simulink model "RobustFormationControl_FractionalModel_under_Dis"  (R2023a)
settings: Solver=ode3  StartTime=0.0  StopTime=30  FixedStep=0.0001  RelTol=1e-3
InitFcn:
  | % close all;
  | % clear all;
  | % clc;
  | % System & Qaudrotor Parameters
  | %==============================
  | m = 0.486;                                         % Quadrotor Mass ( kg )
  | 
  | L = 0.25;                                         % Length of the arm ( m )
  | % L = 0.25;                                         % Length of the arm ( m )
  | 
  | Ixx = 4.856e-03; Iyy = 4.856e-03; Izz = 8.801e-03; % The moments of inertia around x,y and z axes respectively ( kg.m^2 )
  | % Ixx = 3.8278e-03; Iyy = 3.8278e-03; Izz = 7.6566e-03; % The moments of inertia around x,y and z axes respectively ( kg.m^2 )
  | 
  | Jr = 2.8385e-5;                                            % The inertia moment of rotor ( kg.m^2 )
  | % Jr = 0;
  | 
  | % Kx=5.5670e-4;
  | % Ky=5.5670e-4;
  | % Kz=6.3540e-4;
  | % kx=0.032;
  | % ky=0.032;
  | % kz=0.048;
  | Kfx = 5.5670e-4; Kfy = 5.5670e-4; Kfz = 6.3540e-4;% The Rotational drag cofficients ( N/rad/s )
  | 
  | % Ktx = 0.032; Kty = 0.032; Ktz = 0.048;               % The linear drag coefficients in x, y, z respectively ( N/m/s )
  | Ktx = 5.5670e-4; Kty =5.5670e-4; Ktz = 6.3540e-4;               % The linear drag coefficients in x, y, z respectively ( N/m/s )
  | 
  | b = 2.923e-05;                                      % The lift coefficient
  | % b = 2.9842e-05;                                      % The lift coefficient
  | 
  | d = 1.12e-06;                                       % The drag coefficient
  | % d = 3.2320e-07;                                       % The drag coefficient
  | 
  | g = 9.81;                                          % The acceleration due to gravity ( m/s^2 )
  | 
  | %-------- The Coefficients of Non-linear Equations of Quadrotor ( Page 11) -------
  | %--------------------------------------------------------------------------------
  | % Rotational Equations
  | %=====================
  | % Coefficients in ( eq1 ) >>..
  | a1 = (Iyy - Izz)/Ixx;
  | b1 = - Jr/Ixx;
  | c1 = - Kfx/Ixx;
  | d1 = L/Ixx;
  | 
  | % Coefficients in ( eq2 ) >>..
  | a2 = (Izz - Ixx)/Iyy;
  | b2 = Jr/Iyy;
  | c2 = - Kfy/Iyy;
  | d2 = L/Iyy;
  | 
  | % Coefficients in ( eq3 ) >>..
  | a3 = (Ixx - Iyy)/Izz;
  | b3 = - Kfz/Izz;
  | c3 = 1/Izz;
  | % c3 = d/Izz;
  | 
  | % Translational Equations
  | %========================
  | % Coefficients in ( eq4 ) >>..
  | ... (+151 lines)
libraries: fod x135, eeStairGenerator x5
(part 5 of 10)

== system RobustFormationControl_FractionalModel_under_Dis/Fractional Leader with four followers/Follower 4 System/Follower 2 Quadrotor Model/Control Module1/Subsystem1 ==
  x1 : Inport
  x2 : Inport  Port=2
  x3 : Inport  Port=3
  x4 : Inport  Port=4
  x5 : Inport  Port=5
  x6 : Inport  Port=6
  x7 : Inport  Port=7
  x8 : Inport  Port=8
  x9 : Inport  Port=9
  x10 : Inport  Port=10
  x11 : Inport  Port=11
  x12 : Inport  Port=12
  xd1 : Inport  Port=13
  xd2 : Inport  Port=14
  xd3 : Inport  Port=15
  xd4 : Inport  Port=16
  xd5 : Inport  Port=17
  xd6 : Inport  Port=18
  xL : Inport  Port=19
  dX : Inport  Port=20
  yL : Inport  Port=21
  dY : Inport  Port=22
  zL : Inport  Port=23
  dZ : Inport  Port=24
  Subsystem : Subsystem
  Subsystem1 : Subsystem
  Subsystem2 : Subsystem
  Subsystem3 : Subsystem
  Subsystem4 : Subsystem
  Subsystem6 : Subsystem
  S2 : Outport  VectorParamsAs1DForOutWhenUnconnected=off
  S4 : Outport  Port=2  VectorParamsAs1DForOutWhenUnconnected=off
  S6 : Outport  Port=3  VectorParamsAs1DForOutWhenUnconnected=off
  S8 : Outport  Port=4  VectorParamsAs1DForOutWhenUnconnected=off
  S10 : Outport  Port=5  VectorParamsAs1DForOutWhenUnconnected=off
  S12 : Outport  Port=6  VectorParamsAs1DForOutWhenUnconnected=off
  wires:
  x1/1 -> [x1]
  x2/1 -> [x2]
  x3/1 -> [x3]
  x4/1 -> [x4]
  x5/1 -> [x5]
  x6/1 -> [x6]
  x7/1 -> [x7]
  x8/1 -> [x8]
  x9/1 -> [x9]
  x10/1 -> [x10]
  x11/1 -> [x11]
  x12/1 -> [x12]
  xd1/1 -> [xd1]
  dY/1 -> [dY]
  xd2/1 -> [xd2]
  xd3/1 -> [xd3]
  xd4/1 -> [xd4]
  xd5/1 -> [xd5]
  xd6/1 -> [xd6]
  xL/1 -> [xL]
  dX/1 -> [dX]
  yL/1 -> [yL]
  zL/1 -> [zL]
  dZ/1 -> [dZ]
  [x1] -> Subsystem/1(x1)
  [xd1] -> Subsystem/2(xd1)
  [x2] -> Subsystem/3(x2)
  [xd2] -> Subsystem/4(xd2)
  Subsystem/1(S2) -> S2/1
  [xd4] -> Subsystem6/4(xd4)
  [x3] -> Subsystem6/1(x3)
  [x4] -> Subsystem6/3(x4)
  [xd3] -> Subsystem6/2(xd3)
  [xd6] -> Subsystem1/4(xd6)
  [x5] -> Subsystem1/1(x5)
  [x6] -> Subsystem1/3(x6)
  [xd5] -> Subsystem1/2(xd5)
  Subsystem6/1(S4) -> S4/1
  Subsystem1/1(S6) -> S6/1
  [x9] -> Subsystem2/2(x9)
  [x10] -> Subsystem2/3(x10)
  [yL] -> Subsystem2/1(yL)
  [dY] -> Subsystem2/4(dY)
  Subsystem2/1(S10) -> S10/1
  [zL] -> Subsystem4/1(zL)
  [x8] -> Subsystem3/3(x8)
  Subsystem4/1(S12) -> S12/1
  [x12] -> Subsystem4/3(x12)
  Subsystem3/1(S8) -> S8/1
  [dZ] -> Subsystem4/4(dZ)
  [x11] -> Subsystem4/2(x11)
  [x7] -> Subsystem3/2(x7)
  [dX] -> Subsystem3/4(dX)
  [xL] -> Subsystem3/1(xL)

== system RobustFormationControl_FractionalModel_under_Dis/Fractional Leader with four followers/Follower 4 System/Follower 2 Quadrotor Model/Control Module1/Subsystem10 ==
  x1 : Inport
  x3 : Inport  Port=2
  x11 : Inport  Port=3
  x12 : Inport  Port=4
  zL : Inport  Port=5
  dZ : Inport  Port=6
  S12 : Inport  Port=7
  Constant1 : Constant
  Divide1 : Product  Inputs=*/
  Divide2 : Product  Inputs=**  RndMeth=Zero  SaturateOnIntegerOverflow=on
  Gain : Gain  Commented=on  Gain=b6
  Product1 : Product
  Product2 : Product
  Subsystem : Subsystem
  Subsystem1 : Subsystem
  Subsystem2 : Subsystem
  Sum2 : Sum  Inputs=+++
  Trigonometric Function1 : Trigonometry  Operator=cos
  Trigonometric Function2 : Trigonometry  Operator=cos
  U1 : Outport  VectorParamsAs1DForOutWhenUnconnected=off
  wires:
  S12/1 -> [S12]
  dZ/1 -> [dZ]
  zL/1 -> [zL]
  x3/1 -> [x3]
  Sum2/1 -> Product2/2
  Product2/1 -> U1/1
  x11/1 -> [x11]
  x12/1 -> [x12]
  x1/1 -> [x1]
  [x11] -> Subsystem/2(x11)
  [x12] -> Subsystem1/1(x12)
  [zL] -> Subsystem1/2(zL)
  [zL] -> Subsystem/1(zL)
  [dZ] -> Subsystem/4(dZ)
  [x12] -> Subsystem/3(x12)
  [S12] -> Subsystem/5(S12)
  [x11] -> Subsystem2/2(x11)
  [S12] -> Subsystem2/5(S12)
  [x12] -> Subsystem2/3(x12)
  [zL] -> Subsystem2/1(zL)
  [dZ] -> Subsystem2/4(dZ)
  Subsystem/1(D2) -> Sum2/2
  Subsystem2/1(D3) -> Sum2/3
  Subsystem1/1(D1) -> Sum2/1
  Divide1/1 -> Product2/1
  Constant1/1 -> Divide1/1
  Trigonometric Function2/1 -> Product1/2
  Trigonometric Function1/1 -> Product1/1
  Divide2/1 -> Divide1/2
  Product1/1 -> Divide2/2
  [x1] -> Trigonometric Function1/1
  [x3] -> Trigonometric Function2/1
  [b6D] -> Divide2/1
  [dZ] -> Subsystem1/3(dZ)

== system RobustFormationControl_FractionalModel_under_Dis/Fractional Leader with four followers/Follower 4 System/Follower 2 Quadrotor Model/Control Module1/Subsystem2 ==
  U1 : Inport
  x9 : Inport  Port=2
  x10 : Inport  Port=3
  yL : Inport  Port=4
  dY : Inport  Port=5
  S10 : Inport  Port=6
  Constant1 : Constant
  Divide1 : Product  Inputs=*/
  Divide2 : Product  Inputs=**  RndMeth=Zero  SaturateOnIntegerOverflow=on
  Gain1 : Gain  Commented=on  Gain=b4
  Product2 : Product
  Subsystem3 : Subsystem
  Subsystem4 : Subsystem
  Subsystem5 : Subsystem
  Sum1 : Sum  Inputs=+++
  Uy : Outport  VectorParamsAs1DForOutWhenUnconnected=off
  wires:
  S10/1 -> [S10]
  dY/1 -> [dY]
  yL/1 -> [yL]
  Product2/1 -> Uy/1
  x9/1 -> [x9]
  x10/1 -> [x10]
  U1/1 -> [U1]
  Divide1/1 -> Product2/1
  Constant1/1 -> Divide1/1
  [b5D] -> Divide2/1
  [U1] -> Divide2/2
  Divide2/1 -> Divide1/2
  [dY] -> Subsystem4/3(dY)
  [dY] -> Subsystem3/4(dY)
  Subsystem4/1(D1) -> Sum1/1
  Subsystem5/1(D3) -> Sum1/3
  [yL] -> Subsystem5/1(yL)
  Subsystem3/1(D2) -> Sum1/2
  [dY] -> Subsystem5/4(dY)
  [x9] -> Subsystem3/2(x9)
  [yL] -> Subsystem3/1(yL)
  [yL] -> Subsystem4/2(yL)
  [S10] -> Subsystem3/5(S10)
  [x9] -> Subsystem5/2(x9)
  [x10] -> Subsystem5/3(x10)
  [x10] -> Subsystem4/1(x10)
  [x10] -> Subsystem3/3(x10)
  [S10] -> Subsystem5/5(S10)
  Sum1/1 -> Product2/2

== system RobustFormationControl_FractionalModel_under_Dis/Fractional Leader with four followers/Follower 4 System/Follower 2 Quadrotor Model/Control Module1/Subsystem4 ==
  x1 : Inport
  x2 : Inport  Port=2
  x4 : Inport  Port=3
  x6 : Inport  Port=4
  xd1 : Inport  Port=5
  xd2 : Inport  Port=6
  S2 : Inport  Port=7
  Omega : Inport  Port=8
  Constant : Constant
  Constant3 : Constant  Value=d1
  Derivative : Derivative
  Divide : Product  Inputs=*/
  Product2 : Product
  Subsystem : Subsystem
  Subsystem1 : Subsystem
  Subsystem2 : Subsystem
  Sum2 : Sum  Inputs=+++
  U2 : Outport  VectorParamsAs1DForOutWhenUnconnected=off
  wires:
  Constant/1 -> Divide/1
  Constant3/1 -> Divide/2
  S2/1 -> [S2]
  xd2/1 -> [xd2], Derivative/1
  Derivative/1 -> [xdDot2]
  xd1/1 -> [xd1]
  x2/1 -> [x2]
  Sum2/1 -> Product2/2
  Divide/1 -> Product2/1
  Product2/1 -> U2/1
  x4/1 -> [x4]
  x6/1 -> [x6]
  x1/1 -> [x1]
  [x1] -> Subsystem/1(x1)
  [x4] -> Subsystem1/1(x4)
  [x6] -> Subsystem1/2(x6)
  [x2] -> Subsystem1/3(x2)
  Omega/1 -> Subsystem1/4(Omega)
  [xdDot2] -> Subsystem1/5(xd2)
  [xd1] -> Subsystem/2(xd1)
  [xd2] -> Subsystem/4(xd2)
  [x2] -> Subsystem/3(x2)
  [S2] -> Subsystem/5(S2)
  [xd1] -> Subsystem2/2(xd1)
  [S2] -> Subsystem2/5(S2)
  [x2] -> Subsystem2/3(x2)
  [x1] -> Subsystem2/1(x1)
  [xd2] -> Subsystem2/4(xd2)
  Subsystem1/1(D1) -> Sum2/1
  Subsystem/1(D2) -> Sum2/2
  Subsystem2/1(D3) -> Sum2/3

== system RobustFormationControl_FractionalModel_under_Dis/Fractional Leader with four followers/Follower 4 System/Follower 2 Quadrotor Model/Control Module1/Subsystem5 ==
  x5 : Inport
  x2 : Inport  Port=2
  x4 : Inport  Port=3
  x6 : Inport  Port=4
  xd5 : Inport  Port=5
  xd6 : Inport  Port=6
  S6 : Inport  Port=7
  Constant : Constant
  Constant3 : Constant  Value=c3
  Derivative : Derivative
  Divide : Product  Inputs=*/
  Product2 : Product
  Subsystem : Subsystem
  Subsystem1 : Subsystem
  Subsystem2 : Subsystem
  Sum2 : Sum  Inputs=+++
  U4 : Outport  VectorParamsAs1DForOutWhenUnconnected=off
  wires:
  Constant/1 -> Divide/1
  Constant3/1 -> Divide/2
  S6/1 -> [S6]
  xd6/1 -> [xd6], Derivative/1
  Derivative/1 -> [xdDot6]
  xd5/1 -> [xd5]
  x2/1 -> [x2]
  Sum2/1 -> Product2/2
  Divide/1 -> Product2/1
  Product2/1 -> U4/1
  x4/1 -> [x4]
  x6/1 -> [x6]
  x5/1 -> [x5]
  [x5] -> Subsystem/1(x5)
  [x4] -> Subsystem1/1(x4)
  [x6] -> Subsystem1/2(x6)
  [x2] -> Subsystem1/3(x2)
  [xdDot6] -> Subsystem1/4(xd6)
  [xd5] -> Subsystem/2(xd5)
  [xd6] -> Subsystem/4(xd6)
  [x6] -> Subsystem/3(x6)
  [S6] -> Subsystem/5(S4)
  [xd5] -> Subsystem2/2(xd5)
  [S6] -> Subsystem2/5(S6)
  [x6] -> Subsystem2/3(x6)
  [x5] -> Subsystem2/1(x5)
  [xd6] -> Subsystem2/4(xd6)
  Subsystem/1(D2) -> Sum2/2
  Subsystem2/1(D3) -> Sum2/3
  Subsystem1/1(D1) -> Sum2/1

== system RobustFormationControl_FractionalModel_under_Dis/Fractional Leader with four followers/Follower 4 System/Follower 2 Quadrotor Model/Control Module1/Subsystem6 ==
  U1 : Inport
  x7 : Inport  Port=2
  x8 : Inport  Port=3
  xL : Inport  Port=4
  dX : Inport  Port=5
  S8 : Inport  Port=6
  Constant1 : Constant
  Divide1 : Product  Inputs=*/
  Divide2 : Product  Inputs=**  RndMeth=Zero  SaturateOnIntegerOverflow=on
  Gain1 : Gain  Commented=on  Gain=b4
  Product2 : Product
  Subsystem3 : Subsystem
  Subsystem4 : Subsystem
  Subsystem5 : Subsystem
  Sum1 : Sum  Inputs=+++
  Ux : Outport  VectorParamsAs1DForOutWhenUnconnected=off
  wires:
  S8/1 -> [S8]
  dX/1 -> [dX]
  xL/1 -> [xL]
  Product2/1 -> Ux/1
  x7/1 -> [x7]
  x8/1 -> [x8]
  U1/1 -> [U1]
  Divide1/1 -> Product2/1
  Constant1/1 -> Divide1/1
  [b4D] -> Divide2/1
  [U1] -> Divide2/2
  Divide2/1 -> Divide1/2
  [dX] -> Subsystem4/3(dX)
  [dX] -> Subsystem3/4(dX)
  Subsystem4/1(D1) -> Sum1/1
  Subsystem5/1(D3) -> Sum1/3
  [xL] -> Subsystem5/1(xL)
  Subsystem3/1(D2) -> Sum1/2
  [dX] -> Subsystem5/4(dX)
  [x7] -> Subsystem3/2(x7)
  [xL] -> Subsystem3/1(xL)
  [xL] -> Subsystem4/2(xL)
  [S8] -> Subsystem3/5(S8)
  [x7] -> Subsystem5/2(x7)
  [x8] -> Subsystem5/3(x8)
  [x8] -> Subsystem4/1(x8)
  [x8] -> Subsystem3/3(x8)
  [S8] -> Subsystem5/5(S8)
  Sum1/1 -> Product2/2

== system RobustFormationControl_FractionalModel_under_Dis/Fractional Leader with four followers/Follower 4 System/Follower 2 Quadrotor Model/Control Module1/Subsystem8 ==
  x3 : Inport
  x2 : Inport  Port=2
  x4 : Inport  Port=3
  x6 : Inport  Port=4
  xd3 : Inport  Port=5
  xd4 : Inport  Port=6
  S4 : Inport  Port=7
  Omega : Inport  Port=8
  Constant : Constant
  Constant3 : Constant  Value=d2
  Derivative : Derivative
  Divide : Product  Inputs=*/
  Product2 : Product
  Subsystem : Subsystem
  Subsystem1 : Subsystem
  Subsystem2 : Subsystem
  Sum2 : Sum  Inputs=+++
  U3 : Outport  VectorParamsAs1DForOutWhenUnconnected=off
  wires:
  Constant/1 -> Divide/1
  Constant3/1 -> Divide/2
  S4/1 -> [S4]
  xd4/1 -> [xd4], Derivative/1
  Derivative/1 -> [xdDot4]
  xd3/1 -> [xd3]
  x2/1 -> [x2]
  Sum2/1 -> Product2/2
  Divide/1 -> Product2/1
  Product2/1 -> U3/1
  x4/1 -> [x4]
  x6/1 -> [x6]
  x3/1 -> [x3]
  [x3] -> Subsystem/1(x3)
  [x4] -> Subsystem1/1(x4)
  [x6] -> Subsystem1/2(x6)
  [x2] -> Subsystem1/3(x2)
  Omega/1 -> Subsystem1/4(Omega)
  [xdDot4] -> Subsystem1/5(xd4)
  [xd3] -> Subsystem/2(xd3)
  [xd4] -> Subsystem/4(xd4)
  [x4] -> Subsystem/3(x4)
  [S4] -> Subsystem/5(S4)
  [xd3] -> Subsystem2/2(xd3)
  [S4] -> Subsystem2/5(S4)
  [x4] -> Subsystem2/3(x4)
  [x3] -> Subsystem2/1(x3)
  [xd4] -> Subsystem2/4(xd4)
  Subsystem/1(D2) -> Sum2/2
  Subsystem2/1(D3) -> Sum2/3
  Subsystem1/1(D1) -> Sum2/1

== system RobustFormationControl_FractionalModel_under_Dis/Fractional Leader with four followers/Follower 4 System/Follower 2 Quadrotor Model/Quadrotor Dynamic System/Rotational System ==
  U2 : Inport
  U3 : Inport  Port=2
  U4 : Inport  Port=3
  Omega : Inport  Port=4
  Equation1 : Subsystem
  Equation2 : Subsystem
  Equation3 : Subsystem
  Phi or x1 : Outport  VectorParamsAs1DForOutWhenUnconnected=off
  Theta or x3 : Outport  Port=2  VectorParamsAs1DForOutWhenUnconnected=off
  Psi or x5 : Outport  Port=3  VectorParamsAs1DForOutWhenUnconnected=off
  x2 : Outport  Port=4  VectorParamsAs1DForOutWhenUnconnected=off
  x4 : Outport  Port=5  VectorParamsAs1DForOutWhenUnconnected=off
  x6 : Outport  Port=6  VectorParamsAs1DForOutWhenUnconnected=off
  wires:
  Equation1/1(x1 = Phi) -> Phi or x1/1
  Equation3/1(x5 =Psi) -> Psi or x5/1
  U2/1 -> Equation1/3(U2)
  U3/1 -> Equation2/3(U3)
  Equation3/2(x6) -> Equation2/2(x6), x6/1, Equation1/2(x6)
  Equation2/1(x3 =Theta) -> Theta or x3/1
  U4/1 -> Equation3/3(U4)
  Omega/1 -> Equation2/4(Omega), Equation1/4(Omega)
  Equation1/2(x2) -> x2/1, Equation2/1(x2), Equation3/1(x2)
  Equation2/2(x4) -> x4/1, Equation3/2(x4), Equation1/1(x4)

== system RobustFormationControl_FractionalModel_under_Dis/Fractional Leader with four followers/Follower 4 System/Follower 2 Quadrotor Model/Quadrotor Dynamic System/Translational System ==
  U1 : Inport
  Ux : Inport  Port=2
  Uy : Inport  Port=3
  x1 : Inport  Port=4
  x3 : Inport  Port=5
  Equation4 : Subsystem
  Equation5 : Subsystem
  Equation6 : Subsystem
  x or x7 : Outport  VectorParamsAs1DForOutWhenUnconnected=off
  y or x9 : Outport  Port=2  VectorParamsAs1DForOutWhenUnconnected=off
  z or x11 : Outport  Port=3  VectorParamsAs1DForOutWhenUnconnected=off
  xdot or x8 : Outport  Port=4  VectorParamsAs1DForOutWhenUnconnected=off
  ydot or x10 : Outport  Port=5  VectorParamsAs1DForOutWhenUnconnected=off
  zdot or x12 : Outport  Port=6  VectorParamsAs1DForOutWhenUnconnected=off
  wires:
  Ux/1 -> Equation4/2(Ux)
  Uy/1 -> Equation5/2(Uy)
  x1/1 -> Equation6/2(x1)
  x3/1 -> Equation6/3(x3)
  Equation5/1(x9 = y) -> y or x9/1
  Equation6/1(x11 = z) -> z or x11/1
  Equation4/1(x7 = x) -> x or x7/1
  U1/1 -> Equation6/1(U1), Equation5/1(U1), Equation4/1(U1)
  Equation4/2(x8 = xdot) -> xdot or x8/1
  Equation5/2(x10 = ydot) -> ydot or x10/1
  Equation6/2(x12 = zdot) -> zdot or x12/1

== system RobustFormationControl_FractionalModel_under_Dis/Fractional Leader with four followers/Fractional Model of the Leader/Fractional Model/Control Module1/Desired System ==
  ft : Inport
  Derivative : Derivative
  Derivative1 : Derivative
  Derivative2 : Derivative
  Desired Values : Subsystem
  Fractional operator{,1..8} (9 alike) : fod/Fractional operator  Tag=Fractional operator  K=1  gam=0.5  ww=[0.001, 1000]  n=5
      settings: SourceProductName=FOMCON Toolbox
  xd1 : Outport  VectorParamsAs1DForOutWhenUnconnected=off
  xd2 : Outport  Port=2  VectorParamsAs1DForOutWhenUnconnected=off
  xd3 : Outport  Port=3  VectorParamsAs1DForOutWhenUnconnected=off
  xd4 : Outport  Port=4  VectorParamsAs1DForOutWhenUnconnected=off
  xd5 : Outport  Port=5  VectorParamsAs1DForOutWhenUnconnected=off
  xd6 : Outport  Port=6  VectorParamsAs1DForOutWhenUnconnected=off
  xfd7 : Outport  Port=7  VectorParamsAs1DForOutWhenUnconnected=off
  xfd8 : Outport  Port=8  VectorParamsAs1DForOutWhenUnconnected=off
  xfd9 : Outport  Port=9  VectorParamsAs1DForOutWhenUnconnected=off
  xfd10 : Outport  Port=10  VectorParamsAs1DForOutWhenUnconnected=off
  xfd11 : Outport  Port=11  VectorParamsAs1DForOutWhenUnconnected=off
  xfd12 : Outport  Port=12  VectorParamsAs1DForOutWhenUnconnected=off
  xfd13 : Outport  Port=13  VectorParamsAs1DForOutWhenUnconnected=off
  xfd14 : Outport  Port=14  VectorParamsAs1DForOutWhenUnconnected=off
  xfd15 : Outport  Port=15  VectorParamsAs1DForOutWhenUnconnected=off
  xfd16 : Outport  Port=16  VectorParamsAs1DForOutWhenUnconnected=off
  xfd17 : Outport  Port=17  VectorParamsAs1DForOutWhenUnconnected=off
  xfd18 : Outport  Port=18  VectorParamsAs1DForOutWhenUnconnected=off
  wires:
  Fractional operator8/1 -> xfd18/1
  Derivative/1 -> xd6/1
  Fractional operator5/1 -> xfd14/1
  Fractional operator4/1 -> xfd13/1, Fractional operator5/1
  Fractional operator/1 -> Fractional operator1/1, xfd8/1
  Fractional operator3/1 -> xfd12/1, Fractional operator4/1
  [Yd] -> xfd11/1, Fractional operator3/1
  [Xd] -> xfd7/1, Fractional operator/1
  Derivative1/1 -> xd2/1
  [Psi_d] -> Derivative/1, xd5/1
  [Zd] -> xfd15/1, Fractional operator6/1
  Fractional operator2/1 -> xfd10/1
  Fractional operator7/1 -> xfd17/1, Fractional operator8/1
  [Phi_d] -> Derivative1/1, xd1/1
  Fractional operator1/1 -> Fractional operator2/1, xfd9/1
  Fractional operator6/1 -> xfd16/1, Fractional operator7/1
  ft/1 -> Desired Values/1(ft)
  Desired Values/4(Xd) -> [xd]
  Desired Values/5(Yd) -> [yd]
  Desired Values/6(Zd) -> [zd]
  Desired Values/3(Psi_d) -> [Psi_d]
  Derivative2/1 -> xd4/1
  Desired Values/1(Phi_d) -> [Phi_d]
  Desired Values/2(Theta_d) -> [Theta_d]
  [Theta_d] -> Derivative2/1, xd3/1

== system RobustFormationControl_FractionalModel_under_Dis/Fractional Leader with four followers/Fractional Model of the Leader/Fractional Model/Control Module1/Omega Equations ==
  U1 : Inport
  U2 : Inport  Port=2
  U3 : Inport  Port=3
  U4 : Inport  Port=4
  Add1 : Sum  Inputs=+--
  Add2 : Sum  Inputs=+++
  Add3 : Sum  Inputs=++-
  Add5 : Sum  Inputs=+-+
  Control Inputs : Subsystem
  Gain11 : Gain  Gain=1/(4*b)
  Gain12 : Gain  Gain=1/(4*d)
  Gain7 : Gain  Gain=1/(2*b)
  Gain8 : Gain  Gain=1/(2*b)
  Omega : Outport  VectorParamsAs1DForOutWhenUnconnected=off
  wires:
  Add5/1 -> Control Inputs/1(w1_sqt)
  Add1/1 -> Control Inputs/2(w2_sqt)
  Add2/1 -> Control Inputs/3(w3_sqt)
  Gain11/1 -> Add5/1, Add3/1, Add2/1, Add1/1
  Gain12/1 -> Add5/3, Add2/3, Add3/3, Add1/3
  Gain7/1 -> Add5/2, Add2/2
  Gain8/1 -> Add3/2, Add1/2
  U4/1 -> Gain12/1
  U1/1 -> Gain11/1
  U3/1 -> Gain7/1
  U2/1 -> Gain8/1
  Add3/1 -> Control Inputs/4(w4_sqt)
  Control Inputs/1(Omega) -> Omega/1

== system RobustFormationControl_FractionalModel_under_Dis/Fractional Leader with four followers/Fractional Model of the Leader/Fractional Model/Control Module1/Subsystem ==
  Ux : Inport
  Uy : Inport  Port=2
  Psi_d : Inport  Port=3
  Subsystem : Subsystem
  Subsystem1 : Subsystem
  Phi_d : Outport  VectorParamsAs1DForOutWhenUnconnected=off
  Theta_d : Outport  Port=2  VectorParamsAs1DForOutWhenUnconnected=off
  wires:
  Ux/1 -> Subsystem1/1(Ux), Subsystem/1(Ux)
  Uy/1 -> Subsystem1/2(Uy), Subsystem/2(Uy)
  Psi_d/1 -> Subsystem1/3(Psi_d), Subsystem/3(Psi_d)
  Subsystem/1(Phi_d) -> Subsystem1/4(Phi_d), Phi_d/1
  Subsystem1/1(Theta_d) -> Theta_d/1

== system RobustFormationControl_FractionalModel_under_Dis/Fractional Leader with four followers/Fractional Model of the Leader/Fractional Model/Control Module1/Subsystem1 ==
  x1 : Inport
  x2 : Inport  Port=2
  x3 : Inport  Port=3
  x4 : Inport  Port=4
  x5 : Inport  Port=5
  x6 : Inport  Port=6
  xd1 : Inport  Port=7
  xd2 : Inport  Port=8
  xd3 : Inport  Port=9
  xd4 : Inport  Port=10
  xd5 : Inport  Port=11
  xd6 : Inport  Port=12
  Subsystem : Subsystem  Commented=on
  Subsystem1 : Subsystem
  Subsystem2 : Subsystem
  Subsystem3 : Subsystem
  Subsystem5 : Subsystem  Commented=on
  Subsystem7 : Subsystem  Commented=on
  S2 : Outport  VectorParamsAs1DForOutWhenUnconnected=off
  S4 : Outport  Port=2  VectorParamsAs1DForOutWhenUnconnected=off
  S6 : Outport  Port=3  VectorParamsAs1DForOutWhenUnconnected=off
  wires:
  x1/1 -> [x1]
  x2/1 -> [x2]
  x3/1 -> [x3]
  x4/1 -> [x4]
  x5/1 -> [x5]
  x6/1 -> [x6]
  xd1/1 -> [xd1]
  xd2/1 -> [xd2]
  xd3/1 -> [xd3]
  xd4/1 -> [xd4]
  xd5/1 -> [xd5]
  xd6/1 -> [xd6]
  [x1] -> Subsystem3/1(x1)
  [xd1] -> Subsystem3/2(xd1)
  [x2] -> Subsystem3/3(x2)
  [xd2] -> Subsystem3/4(xd2)
  Subsystem3/1(S2) -> S2/1
  [xd4] -> Subsystem1/4(xd4)
  [x3] -> Subsystem1/1(x3)
  [x4] -> Subsystem1/3(x4)
  [xd3] -> Subsystem1/2(xd3)
  [xd6] -> Subsystem2/4(xd6)
  [x5] -> Subsystem2/1(x5)
  [x6] -> Subsystem2/3(x6)
  [xd5] -> Subsystem2/2(xd5)
  Subsystem1/1(S4) -> S4/1
  Subsystem2/1(S6) -> S6/1

== system RobustFormationControl_FractionalModel_under_Dis/Fractional Leader with four followers/Fractional Model of the Leader/Fractional Model/Control Module1/Subsystem2 ==
  x1 : Inport
  x3 : Inport  Port=2
  xf15 : Inport  Port=3
  xf16 : Inport  Port=4
  xf17 : Inport  Port=5
  xf18 : Inport  Port=6
  xfd15 : Inport  Port=7
  xfd16 : Inport  Port=8
  xfd17 : Inport  Port=9
  xfd18 : Inport  Port=10
  S12 : Inport  Port=11
  Constant : Constant
  Constant1 : Constant  Value=q18
  Constant2 : Constant  Value=g
  Divide : Product  Inputs=*/
  Divide1 : Product  Inputs=**  RndMeth=Zero  SaturateOnIntegerOverflow=on
  Divide2 : Product  Inputs=**  RndMeth=Zero  SaturateOnIntegerOverflow=on
  Fractional operator{,1..3} (4 alike) : fod/Fractional operator  Tag=Fractional operator  K=1  gam=0.5  ww=[0.001, 1000]  n=5
      settings: SourceProductName=FOMCON Toolbox
  Gain1 : Gain  Gain=gZ
  Gain2 : Gain  Gain=sZ
  Gain4 : Gain  Gain=q18
  Gain5 : Gain  Gain=q15
  Gain6 : Gain  Gain=q16
  Gain7 : Gain  Gain=q17
  Gain8 : Gain  Commented=on  Gain=b6
  Gain9 : Gain  Commented=on  Gain=a6
  Product : Product
  Product1 : Product
  Product2 : Product
  Subsystem2 : Subsystem
  Sum : Sum  Inputs=+--
  Sum1 : Sum  Inputs=+-
  Sum2 : Sum  Inputs=-------
  Sum3 : Sum  Inputs=+-
  Sum4 : Sum  Inputs=+-
  Tanh : Trigonometry  Operator=tanh
  Trigonometric Function1 : Trigonometry  Operator=cos
  Trigonometric Function2 : Trigonometry  Operator=cos
  U1 : Outport  VectorParamsAs1DForOutWhenUnconnected=off
  wires:
  Constant/1 -> Divide/1
  Product/1 -> Divide/2
  x1/1 -> Trigonometric Function1/1
  x3/1 -> Trigonometric Function2/1
  Trigonometric Function2/1 -> Product1/2
  Trigonometric Function1/1 -> Product1/1
  Divide1/1 -> Product/1
  Constant1/1 -> Product/2
  S12/1 -> [S12]
  xf16/1 -> [xf16]
  [S12] -> Tanh/1, Gain2/1
  Tanh/1 -> Gain1/1
  [xf16] -> Sum1/1
  [xfd15] -> Sum1/2
  Sum1/1 -> Gain5/1
  Gain1/1 -> Sum2/1
  Gain2/1 -> Sum2/2
  Sum2/1 -> Product2/2
  Divide/1 -> Product2/1
  Product2/1 -> U1/1
  xf17/1 -> [xf17]
  xf18/1 -> [xf18]
  xfd15/1 -> Subsystem2/5(x15fd), Fractional operator/1
  Fractional operator/1 -> [xfd15]
  Fractional operator1/1 -> [xfd16]
  xfd16/1 -> Subsystem2/6(x16fd), Fractional operator1/1
  Fractional operator2/1 -> [xfd17]
  xfd17/1 -> Subsystem2/7(x17fd), Fractional operator2/1
  Fractional operator3/1 -> [xfd18]
  xfd18/1 -> Subsystem2/8(x18fd), Fractional operator3/1
  [xfd18] -> Sum/3
  Sum/1 -> Gain4/1
  Constant2/1 -> Sum/2
  Divide2/1 -> Sum/1
  [xf17] -> Divide2/1
  Gain5/1 -> Sum2/3
  Sum3/1 -> Gain6/1
  [xfd16] -> Sum3/2
  [xf17] -> Sum3/1
  Gain6/1 -> Sum2/4
  Sum4/1 -> Gain7/1
  [xfd17] -> Sum4/2
  [xf18] -> Sum4/1
  Gain7/1 -> Sum2/5
  Gain4/1 -> Sum2/6
  [b6D] -> Divide1/1
  Product1/1 -> Divide1/2
  [a6D] -> Divide2/2
  Subsystem2/1(D) -> Sum2/7
  xf15/1 -> [xf15]
  [S12] -> Subsystem2/9(S12)
  [xf15] -> Subsystem2/1(x15f)
  [xf16] -> Subsystem2/2(x16f)
  [xf17] -> Subsystem2/3(x17f)
  [xf18] -> Subsystem2/4(x18f)

== system RobustFormationControl_FractionalModel_under_Dis/Fractional Leader with four followers/Fractional Model of the Leader/Fractional Model/Control Module1/Subsystem3 ==
  U1 : Inport
  xf7 : Inport  Port=2
  xf8 : Inport  Port=3
  xf9 : Inport  Port=4
  xf10 : Inport  Port=5
  xfd7 : Inport  Port=6
  xfd8 : Inport  Port=7
  xfd9 : Inport  Port=8
  xfd10 : Inport  Port=9
  S8 : Inport  Port=10
  Constant : Constant
  Constant1 : Constant  Value=q10
  Divide : Product  Inputs=*/
  Divide1 : Product  Inputs=**  RndMeth=Zero  SaturateOnIntegerOverflow=on
  Divide2 : Product  Inputs=**  RndMeth=Zero  SaturateOnIntegerOverflow=on
  Fractional operator{,1..3} (4 alike) : fod/Fractional operator  Tag=Fractional operator  K=1  gam=0.5  ww=[0.001, 1000]  n=5
      settings: SourceProductName=FOMCON Toolbox
  Gain : Gain  Commented=on  Gain=b4
  Gain1 : Gain  Gain=gX
  Gain2 : Gain  Gain=sX
  Gain3 : Gain  Commented=on  Gain=a4
  Gain4 : Gain  Gain=q10
  Gain5 : Gain  Gain=q7
  Gain6 : Gain  Gain=q8
  Gain7 : Gain  Gain=q9
  Product : Product
  Product2 : Product
  Subsystem2 : Subsystem
  Sum{,1,3..4} (4 alike) : Sum  Inputs=+-
  Sum2 : Sum  Inputs=-------
  Tan : Trigonometry  Operator=tanh
  Ux : Outport  VectorParamsAs1DForOutWhenUnconnected=off
  wires:
  xfd8/1 -> Subsystem2/6(x8fd), Fractional operator1/1
  [xf9] -> Sum3/1
  [xfd8] -> Sum3/2
  Divide2/1 -> Sum/1
  Gain4/1 -> Sum2/6
  Gain6/1 -> Sum2/4
  xfd10/1 -> Subsystem2/8(x10fd), Fractional operator3/1
  Fractional operator3/1 -> [xfd10]
  Gain5/1 -> Sum2/3
  Fractional operator1/1 -> [xfd8]
  [xf10] -> Sum4/1
  [xfd9] -> Sum4/2
  Fractional operator/1 -> [xfd7]
  Sum4/1 -> Gain7/1
  Sum1/1 -> Gain5/1
  Sum2/1 -> Product2/2
  Gain2/1 -> Sum2/2
  Divide/1 -> Product2/1
  Gain1/1 -> Sum2/1
  Constant/1 -> Divide/1
  S8/1 -> [S8]
  [xf8] -> Sum1/1
  Product/1 -> Divide/2
  Product2/1 -> Ux/1
  xfd9/1 -> Subsystem2/7(x9fd), Fractional operator2/1
  [S8] -> Tan/1, Gain2/1
  Fractional operator2/1 -> [xfd9]
  xf10/1 -> [xf10]
  Tan/1 -> Gain1/1
  xf9/1 -> [xf9]
  Sum/1 -> Gain4/1
  [xfd7] -> Sum1/2
  [xf9] -> Divide2/2
  Divide1/1 -> Product/1
  Constant1/1 -> Product/2
  Sum3/1 -> Gain6/1
  xfd7/1 -> Subsystem2/5(x7fd), Fractional operator/1
  xf8/1 -> [xf8]
  Gain7/1 -> Sum2/5
  [xfd10] -> Sum/2
  U1/1 -> Divide1/2
  [b4D] -> Divide1/1
  [a4D] -> Divide2/1
  xf7/1 -> [xf7]
  Subsystem2/1(D) -> Sum2/7
  [xf7] -> Subsystem2/1(x7f)
  [xf8] -> Subsystem2/2(x8f)
  [xf9] -> Subsystem2/3(x9f)
  [xf10] -> Subsystem2/4(x10f)
  [S8] -> Subsystem2/9(S2)

== system RobustFormationControl_FractionalModel_under_Dis/Fractional Leader with four followers/Fractional Model of the Leader/Fractional Model/Control Module1/Subsystem4 ==
  x1 : Inport
  x2 : Inport  Port=2
  x4 : Inport  Port=3
  x6 : Inport  Port=4
  xd1 : Inport  Port=5
  xd2 : Inport  Port=6
  S2 : Inport  Port=7
  Omega : Inport  Port=8
  Constant : Constant
  Constant1 : Constant  Value=k2
  Derivative : Derivative
  Derivative1 : Derivative
  Divide : Product  Inputs=*/
  Gain : Gain
  Gain1 : Gain  Gain=qPhi
  Gain2 : Gain  Gain=kPhi
  Gain5 : Gain  Gain=k1
  Gain8 : Gain  Gain=k2
  Math Function : Math  Operator=square  SignedPower=on
  Product{,1..6} (7 alike) : Product
  Subsystem2 : Subsystem
  Sum1 : Sum  Inputs=+-
  Sum2 : Sum  Inputs=-----
  Sum3 : Sum  Inputs=+++-
  Tanh : Trigonometry  Operator=tanh
  U2 : Outport  VectorParamsAs1DForOutWhenUnconnected=off
  wires:
  Constant/1 -> Divide/1
  Product/1 -> Divide/2
  [d1D] -> Product/1
  Constant1/1 -> Product/2
  S2/1 -> [S2]
  xd2/1 -> Subsystem2/4(xd2), Derivative/1
  Derivative/1 -> [xd2]
  Derivative1/1 -> [xd1]
  xd1/1 -> Derivative1/1, Subsystem2/2(xd1)
  x2/1 -> [x2]
  [S2] -> Tanh/1, Gain2/1
  Tanh/1 -> Gain1/1
  [x2] -> Sum1/1
  [xd1] -> Sum1/2
  Sum1/1 -> Gain5/1
  Gain1/1 -> Sum2/1
  Gain2/1 -> Sum2/2
  Gain5/1 -> Sum2/4
  Sum2/1 -> Product2/2
  Divide/1 -> Product2/1
  Product2/1 -> U2/1
  x4/1 -> [x4]
  x6/1 -> [x6]
  [x4] -> Product3/1, Product1/1
  Product6/1 -> Sum3/3
  Product3/1 -> Product6/2
  Omega/1 -> Product3/2
  Product1/1 -> Product4/2
  Math Function/1 -> Product5/2  "x2^2"
  Sum3/1 -> Gain8/1
  [x6] -> Product1/2
  Gain8/1 -> Sum2/3
  [x2] -> Math Function/1
  Product5/1 -> Sum3/2  "c1 x2^2"
  Product4/1 -> Sum3/1  "a1 x4 x6"
  [xd2] -> Sum3/4
  x1/1 -> [x1]
  [x1] -> Subsystem2/1(x1)
  Subsystem2/1(D) -> Gain/1
  [x2] -> Subsystem2/3(x2)
  [S2] -> Subsystem2/5(S2)
  [a1D] -> Product4/1
  [c1D] -> Product5/1
  [b1D] -> Product6/1
  Gain/1 -> Sum2/5

== system RobustFormationControl_FractionalModel_under_Dis/Fractional Leader with four followers/Fractional Model of the Leader/Fractional Model/Control Module1/Subsystem5 ==
  x2 : Inport
  x3 : Inport  Port=2
  x4 : Inport  Port=3
  x6 : Inport  Port=4
  xd3 : Inport  Port=5
  xd4 : Inport  Port=6
  S4 : Inport  Port=7
  Omega : Inport  Port=8
  Constant : Constant
  Constant1 : Constant  Value=k4
  Derivative : Derivative
  Derivative1 : Derivative
  Divide : Product  Inputs=*/
  Gain : Gain
  Gain1 : Gain  Gain=qTheta
  Gain2 : Gain  Gain=kTheta
  Gain5 : Gain  Gain=k3
  Gain8 : Gain  Gain=k4
  Math Function : Math  Operator=square  SignedPower=on
  Product{,1..6} (7 alike) : Product
  Subsystem2 : Subsystem
  Sum1 : Sum  Inputs=+-
  Sum2 : Sum  Inputs=-----
  Sum3 : Sum  Inputs=+++-
  Tanh : Trigonometry  Operator=tanh
  U3 : Outport  VectorParamsAs1DForOutWhenUnconnected=off
  wires:
  Constant/1 -> Divide/1
  Product/1 -> Divide/2
  [d2D] -> Product/1
  Constant1/1 -> Product/2
  S4/1 -> [S4]
  xd4/1 -> Subsystem2/4(xd4), Derivative/1
  Derivative/1 -> [xd4]
  Derivative1/1 -> [xd3]
  xd3/1 -> Subsystem2/2(xd3), Derivative1/1
  x2/1 -> [x2]
  [S4] -> Tanh/1, Gain2/1
  Tanh/1 -> Gain1/1
  [x4] -> Sum1/1
  [xd3] -> Sum1/2
  Sum1/1 -> Gain5/1
  Gain1/1 -> Sum2/1
  Gain2/1 -> Sum2/2
  Gain5/1 -> Sum2/4
  Sum2/1 -> Product2/2
  Divide/1 -> Product2/1
  Product2/1 -> U3/1
  x4/1 -> [x4]
  x6/1 -> [x6]
  [x2] -> Product3/1, Product1/1
  Product6/1 -> Sum3/3
  Product3/1 -> Product6/1
  Omega/1 -> Product3/2
  Sum3/1 -> Gain8/1
  [x6] -> Product1/2
  Gain8/1 -> Sum2/3
  [x4] -> Math Function/1
  Product5/1 -> Sum3/2  "c1 x2^2"
  Product4/1 -> Sum3/1  "a1 x4 x6"
  [xd4] -> Sum3/4
  [a2D] -> Product4/1
  Product1/1 -> Product4/2
  Math Function/1 -> Product5/2  "x2^2"
  [c2D] -> Product5/1
  [b2D] -> Product6/2
  Subsystem2/1(D) -> Gain/1
  x3/1 -> [x3]
  [x3] -> Subsystem2/1(x3)
  [x4] -> Subsystem2/3(x4)
  [S4] -> Subsystem2/5(S4)
  Gain/1 -> Sum2/5

== system RobustFormationControl_FractionalModel_under_Dis/Fractional Leader with four followers/Fractional Model of the Leader/Fractional Model/Control Module1/Subsystem6 ==
  x2 : Inport
  x4 : Inport  Port=2
  x5 : Inport  Port=3
  x6 : Inport  Port=4
  xd5 : Inport  Port=5
  xd6 : Inport  Port=6
  S6 : Inport  Port=7
  Constant : Constant
  Constant1 : Constant  Value=k6
  Derivative : Derivative
  Derivative1 : Derivative
  Divide : Product  Inputs=*/
  Gain : Gain
  Gain1 : Gain  Gain=qPsi
  Gain2 : Gain  Gain=kPsi
  Gain5 : Gain  Gain=k5
  Gain8 : Gain  Gain=k6
  Math Function : Math  Operator=square  SignedPower=on
  Product{,1..4} (5 alike) : Product
  Subsystem2 : Subsystem
  Sum1 : Sum  Inputs=+-
  Sum2 : Sum  Inputs=-----
  Sum3 : Sum  Inputs=++-
  Tanh : Trigonometry  Operator=tanh
  U4 : Outport  VectorParamsAs1DForOutWhenUnconnected=off
  wires:
  Constant/1 -> Divide/1
  Product/1 -> Divide/2
  [c3D] -> Product/1
  Constant1/1 -> Product/2
  S6/1 -> [S6]
  xd6/1 -> Derivative/1, Subsystem2/4(xd6)
  Derivative/1 -> [xd6]
  Derivative1/1 -> [xd5]
  xd5/1 -> Subsystem2/2(xd5), Derivative1/1
  x2/1 -> [x2]
  [S6] -> Tanh/1, Gain2/1
  Tanh/1 -> Gain1/1
  [x6] -> Sum1/1
  [xd5] -> Sum1/2
  Sum1/1 -> Gain5/1
  Gain1/1 -> Sum2/1
  Gain2/1 -> Sum2/2
  Gain5/1 -> Sum2/4
  Sum2/1 -> Product2/2
  Divide/1 -> Product2/1
  Product2/1 -> U4/1
  x4/1 -> [x4]
  x6/1 -> [x6]
  [x2] -> Product1/1
  Product1/1 -> Product3/2
  Math Function/1 -> Product4/2  "x2^2"
  Sum3/1 -> Gain8/1
  [x4] -> Product1/2
  Gain8/1 -> Sum2/3
  [x6] -> Math Function/1
  Product4/1 -> Sum3/2  "c1 x2^2"
  Product3/1 -> Sum3/1  "a1 x4 x6"
  [xd6] -> Sum3/3
  Subsystem2/1(D) -> Gain/1
  x5/1 -> [x5]
  [x5] -> Subsystem2/1(x5)
  [x6] -> Subsystem2/3(x6)
  [S6] -> Subsystem2/5(S6)
  [a3D] -> Product3/1
  [b3D] -> Product4/1
  Gain/1 -> Sum2/5

== system RobustFormationControl_FractionalModel_under_Dis/Fractional Leader with four followers/Fractional Model of the Leader/Fractional Model/Control Module1/Subsystem7 ==
  U1 : Inport
  xf11 : Inport  Port=2
  xf12 : Inport  Port=3
  xf13 : Inport  Port=4
  xf14 : Inport  Port=5
  xfd11 : Inport  Port=6
  xfd12 : Inport  Port=7
  xfd13 : Inport  Port=8
  xfd14 : Inport  Port=9
  S10 : Inport  Port=10
  Constant : Constant
  Constant1 : Constant  Value=q14
  Divide : Product  Inputs=*/
  Divide1 : Product  Inputs=**  RndMeth=Zero  SaturateOnIntegerOverflow=on
  Divide2 : Product  Inputs=**  RndMeth=Zero  SaturateOnIntegerOverflow=on
  Fractional operator{,1..3} (4 alike) : fod/Fractional operator  Tag=Fractional operator  K=1  gam=0.5  ww=[0.001, 1000]  n=5
      settings: SourceProductName=FOMCON Toolbox
  Gain : Gain  Commented=on  Gain=b5
  Gain1 : Gain  Gain=gY
  Gain2 : Gain  Gain=sY
  Gain3 : Gain  Commented=on  Gain=a5
  Gain4 : Gain  Gain=q14
  Gain5 : Gain  Gain=q11
  Gain6 : Gain  Gain=q12
  Gain7 : Gain  Gain=q13
  Product : Product
  Product2 : Product
  Subsystem2 : Subsystem
  Sum{,1,3..4} (4 alike) : Sum  Inputs=+-
  Sum2 : Sum  Inputs=-------
  Tanh : Trigonometry  Operator=tanh
  Uy : Outport  VectorParamsAs1DForOutWhenUnconnected=off
  wires:
  [xfd14] -> Sum/2
  Gain6/1 -> Sum2/4
  Gain4/1 -> Sum2/6
  [xfd12] -> Sum3/2
  [xf13] -> Sum3/1
  Product2/1 -> Uy/1
  S10/1 -> [S10]
  Product/1 -> Divide/2
  Gain1/1 -> Sum2/1
  Divide/1 -> Product2/1
  Gain2/1 -> Sum2/2
  xfd14/1 -> Subsystem2/8(x14fd), Fractional operator3/1
  Sum2/1 -> Product2/2
  Sum4/1 -> Gain7/1
  Sum1/1 -> Gain5/1
  Fractional operator/1 -> [xfd11]
  [xf12] -> Sum1/1
  Gain5/1 -> Sum2/3
  [xfd13] -> Sum4/2
  Constant/1 -> Divide/1
  Divide2/1 -> Sum/1
  U1/1 -> Divide1/2
  [xf14] -> Sum4/1
  [xf13] -> Divide2/2
  [xfd11] -> Sum1/2
  xf13/1 -> [xf13]
  Fractional operator1/1 -> [xfd12]
  Tanh/1 -> Gain1/1
  Sum/1 -> Gain4/1
  xf14/1 -> [xf14]
  [S10] -> Tanh/1, Gain2/1
  Fractional operator2/1 -> [xfd13]
  Fractional operator3/1 -> [xfd14]
  xfd13/1 -> Subsystem2/7(x13fd), Fractional operator2/1
  Gain7/1 -> Sum2/5
  Constant1/1 -> Product/2
  xfd12/1 -> Fractional operator1/1, Subsystem2/6(x12fd)
  Sum3/1 -> Gain6/1
  Divide1/1 -> Product/1
  xf12/1 -> [xf12]
  xfd11/1 -> Subsystem2/5(x11fd), Fractional operator/1
  [b5D] -> Divide1/1
  [a5D] -> Divide2/1
  xf11/1 -> [xf11]
  Subsystem2/1(D) -> Sum2/7
  [xf12] -> Subsystem2/2(x12f)
  [xf11] -> Subsystem2/1(x11f)
  [xf13] -> Subsystem2/3(x13f)
  [xf14] -> Subsystem2/4(x14f)
  [S10] -> Subsystem2/9(S4)

== system RobustFormationControl_FractionalModel_under_Dis/Fractional Leader with four followers/Fractional Model of the Leader/Fractional Model/Control Module1/Subsystem8 ==
  xf7 : Inport
  xf8 : Inport  Port=2
  xf9 : Inport  Port=3
  xf10 : Inport  Port=4
  xf11 : Inport  Port=5
  xf12 : Inport  Port=6
  xf13 : Inport  Port=7
  xf14 : Inport  Port=8
  xf15 : Inport  Port=9
  xf16 : Inport  Port=10
  xf17 : Inport  Port=11
  xf18 : Inport  Port=12
  xfd7 : Inport  Port=13
  xfd8 : Inport  Port=14
  xfd9 : Inport  Port=15
  xfd10 : Inport  Port=16
  xfd11 : Inport  Port=17
  xfd12 : Inport  Port=18
  xfd13 : Inport  Port=19
  xfd14 : Inport  Port=20
  xfd15 : Inport  Port=21
  xfd16 : Inport  Port=22
  xfd17 : Inport  Port=23
  xfd18 : Inport  Port=24
  Subsystem1 : Subsystem
  Subsystem2 : Subsystem
  Subsystem3 : Subsystem
  S8 : Outport  VectorParamsAs1DForOutWhenUnconnected=off
  S10 : Outport  Port=2  VectorParamsAs1DForOutWhenUnconnected=off
  S12 : Outport  Port=3  VectorParamsAs1DForOutWhenUnconnected=off
  wires:
  Subsystem3/1(S8) -> S8/1
  xf12/1 -> [xf12]
  xf11/1 -> [xf11]
  xf9/1 -> [xf9]
  xf8/1 -> [xf8]
  xf16/1 -> [xf16]
  xf14/1 -> [xf14]
  xf10/1 -> [xf10]
  xf7/1 -> [xf7]
  xf13/1 -> [xf13]
  xf15/1 -> [xf15]
  xf17/1 -> [xf17]
  xf18/1 -> [xf18]
  xfd7/1 -> [xfd7]
  xfd8/1 -> [xfd8]
  xfd9/1 -> [xfd9]
  xfd10/1 -> [xfd10]
  xfd11/1 -> [xfd11]
  xfd12/1 -> [xfd12]
  xfd13/1 -> [xfd13]
  xfd14/1 -> [xfd14]
  xfd15/1 -> [xfd15]
  xfd16/1 -> [xfd16]
  xfd17/1 -> [xfd17]
  xfd18/1 -> [xfd18]
  [xf7] -> Subsystem3/1(xf7)
  [xfd7] -> Subsystem3/2(xfd7)
  [xf8] -> Subsystem3/3(xf8)
  [xfd8] -> Subsystem3/4(xfd8)
  [xf9] -> Subsystem3/5(xf9)
  [xfd9] -> Subsystem3/6(xfd9)
  [xf10] -> Subsystem3/7(xf10)
  [xfd10] -> Subsystem3/8(xfd10)
  [xf11] -> Subsystem1/1(xf11)
  [xf14] -> Subsystem1/7(xf14)
  [xfd14] -> Subsystem1/8(xfd14)
  [xfd12] -> Subsystem1/4(xfd12)
  [xfd13] -> Subsystem1/6(xfd13)
  [xf12] -> Subsystem1/3(xf12)
  Subsystem1/1(S10) -> S10/1
  [xfd11] -> Subsystem1/2(xfd11)
  [xf13] -> Subsystem1/5(xf13)
  [xf15] -> Subsystem2/1(xf15)
  [xf18] -> Subsystem2/7(xf18)
  [xfd18] -> Subsystem2/8(xfd18)
  [xfd16] -> Subsystem2/4(xfd16)
  [xfd17] -> Subsystem2/6(xfd17)
  [xf16] -> Subsystem2/3(xf16)
  Subsystem2/1(S12) -> S12/1
  [xfd15] -> Subsystem2/2(xfd15)
  [xf17] -> Subsystem2/5(xf17)

== system RobustFormationControl_FractionalModel_under_Dis/Fractional Leader with four followers/Fractional Model of the Leader/Fractional Model/Quadrotor Dynamic System/Fractional Translational System ==
  U1 : Inport
  Ux : Inport  Port=2
  Uy : Inport  Port=3
  x1 : Inport  Port=4
  x3 : Inport  Port=5
  Equation4 : Subsystem
  Equation5 : Subsystem
  Equation6 : Subsystem
  xf7 : Outport  VectorParamsAs1DForOutWhenUnconnected=off
  xf8 : Outport  Port=2  VectorParamsAs1DForOutWhenUnconnected=off
  xf9 : Outport  Port=3  VectorParamsAs1DForOutWhenUnconnected=off
  xf10 : Outport  Port=4  VectorParamsAs1DForOutWhenUnconnected=off
  xf11 : Outport  Port=5  VectorParamsAs1DForOutWhenUnconnected=off
  xf12 : Outport  Port=6  VectorParamsAs1DForOutWhenUnconnected=off
  xf13 : Outport  Port=7  VectorParamsAs1DForOutWhenUnconnected=off
  xf14 : Outport  Port=8  VectorParamsAs1DForOutWhenUnconnected=off
  xf15 : Outport  Port=9  VectorParamsAs1DForOutWhenUnconnected=off
  xf16 : Outport  Port=10  VectorParamsAs1DForOutWhenUnconnected=off
  xf17 : Outport  Port=11  VectorParamsAs1DForOutWhenUnconnected=off
  xf18 : Outport  Port=12  VectorParamsAs1DForOutWhenUnconnected=off
  wires:
  Ux/1 -> Equation4/2(Ux)
  Uy/1 -> Equation5/2(Uy)
  x1/1 -> Equation6/2(x1)
  x3/1 -> Equation6/3(x3)
  Equation5/1(xf11) -> xf11/1
  Equation6/1(xf15) -> xf15/1
  Equation4/1(xf7) -> xf7/1
  U1/1 -> Equation6/1(U1), Equation5/1(U1), Equation4/1(U1)
  Equation4/2(xf8) -> xf8/1
  Equation4/3(xf9) -> xf9/1
  Equation4/4(xf10) -> xf10/1
  Equation5/4(xf14) -> xf14/1
  Equation5/3(xf13) -> xf13/1
  Equation5/2(xf12) -> xf12/1
  Equation6/4(xf18) -> xf18/1
  Equation6/3(xf17) -> xf17/1
  Equation6/2(xf16) -> xf16/1

== system RobustFormationControl_FractionalModel_under_Dis/Fractional Leader with four followers/Fractional Model of the Leader/Fractional Model/Quadrotor Dynamic System/Rotational System ==
  U2 : Inport
  U3 : Inport  Port=2
  U4 : Inport  Port=3
  Omega : Inport  Port=4
  Equation1 : Subsystem
  Equation2 : Subsystem
  Equation3 : Subsystem
  Phi or x1 : Outport  VectorParamsAs1DForOutWhenUnconnected=off
  Theta or x3 : Outport  Port=2  VectorParamsAs1DForOutWhenUnconnected=off
  Psi or x5 : Outport  Port=3  VectorParamsAs1DForOutWhenUnconnected=off
  x2 : Outport  Port=4  VectorParamsAs1DForOutWhenUnconnected=off
  x4 : Outport  Port=5  VectorParamsAs1DForOutWhenUnconnected=off
  x6 : Outport  Port=6  VectorParamsAs1DForOutWhenUnconnected=off
  wires:
  Equation1/1(x1 = Phi) -> Phi or x1/1
  Equation3/1(x5 =Psi) -> Psi or x5/1
  U2/1 -> Equation1/3(U2)
  U3/1 -> Equation2/3(U3)
  Equation3/2(x6) -> Equation2/2(x6), x6/1, Equation1/2(x6)
  Equation2/1(x3 =Theta) -> Theta or x3/1
  U4/1 -> Equation3/3(U4)
  Omega/1 -> Equation2/4(Omega), Equation1/4(Omega)
  Equation1/2(x2) -> x2/1, Equation2/1(x2), Equation3/1(x2)
  Equation2/2(x4) -> x4/1, Equation3/2(x4), Equation1/1(x4)

== system RobustFormationControl_FractionalModel_under_Dis/Fractional Leader with four followers/Follower 1 System/Follower 1 Quadrotor Model/Control Module1/Omega Equations/Control Inputs ==
  w1_sqt : Inport
  w2_sqt : Inport  Port=2
  w3_sqt : Inport  Port=3
  w4_sqt : Inport  Port=4
  Add4 : Sum  Inputs=+-+-
  Omega : Outport  VectorParamsAs1DForOutWhenUnconnected=off
  wires:
  Add4/1 -> Omega/1
  w1_sqt/1 -> Add4/1
  w2_sqt/1 -> Add4/2
  w3_sqt/1 -> Add4/3
  w4_sqt/1 -> Add4/4

== system RobustFormationControl_FractionalModel_under_Dis/Fractional Leader with four followers/Follower 1 System/Follower 1 Quadrotor Model/Control Module1/Subsystem/Subsystem ==
  Ux : Inport
  Uy : Inport  Port=2
  Psi_d : Inport  Port=3
  Product : Product
  Product1 : Product
  Subtract : Sum  Inputs=+-
  Trigonometric Function : Trigonometry
  Trigonometric Function1 : Trigonometry  Operator=cos
  Trigonometric Function2 : Trigonometry  Operator=asin
  Phi_d : Outport  VectorParamsAs1DForOutWhenUnconnected=off
  wires:
  Product1/1 -> Subtract/2
  Uy/1 -> Product1/2
  Ux/1 -> Product/1
  Trigonometric Function1/1 -> Product1/1
  Psi_d/1 -> Trigonometric Function1/1, Trigonometric Function/1
  Product/1 -> Subtract/1
  Subtract/1 -> Trigonometric Function2/1
  Trigonometric Function/1 -> Product/2
  Trigonometric Function2/1 -> Phi_d/1

== system RobustFormationControl_FractionalModel_under_Dis/Fractional Leader with four followers/Follower 1 System/Follower 1 Quadrotor Model/Control Module1/Subsystem/Subsystem1 ==
  Ux : Inport
  Uy : Inport  Port=2
  Psi_d : Inport  Port=3
  Phi_d : Inport  Port=4
  Constant : Constant
  Divide : Product  Inputs=*/
  Product : Product
  Product1 : Product
  Product2 : Product
  Subtract : Sum
  Trigonometric Function : Trigonometry  Operator=cos
  Trigonometric Function1 : Trigonometry
  Trigonometric Function2 : Trigonometry  Operator=asin
  Trigonometric Function3 : Trigonometry  Operator=cos
  Theta_d : Outport  VectorParamsAs1DForOutWhenUnconnected=off
  wires:
  Product1/1 -> Subtract/2
  Uy/1 -> Product1/2
  Ux/1 -> Product/1
  Trigonometric Function1/1 -> Product1/1
  Psi_d/1 -> Trigonometric Function1/1, Trigonometric Function/1
  Product/1 -> Subtract/1
  Trigonometric Function/1 -> Product/2
  Trigonometric Function2/1 -> Theta_d/1
  Constant/1 -> Divide/1
  Product2/1 -> Trigonometric Function2/1
  Subtract/1 -> Product2/1
  Divide/1 -> Product2/2
  Trigonometric Function3/1 -> Divide/2
  Phi_d/1 -> Trigonometric Function3/1

== system RobustFormationControl_FractionalModel_under_Dis/Fractional Leader with four followers/Follower 1 System/Follower 1 Quadrotor Model/Control Module1/Subsystem1/Subsystem ==
  x1 : Inport
  xd1 : Inport  Port=2
  x2 : Inport  Port=3
  xd2 : Inport  Port=4
  Constant : Constant  Value=p/q
  Constant1 : Constant  Value=gx
  Divide : Product  Inputs=**  RndMeth=Zero  SaturateOnIntegerOverflow=on
  Fractional integrator : fod/Fractional integrator  gam=alpha1(1)  ww=[0.001; 1000]  n=5  nFod=off
      settings: SourceProductName=FOMCON Toolbox
  Fractional integrator1 : fod/Fractional integrator  gam=alpha2(1)  ww=[0.001; 1000]  n=5  nFod=off
      settings: SourceProductName=FOMCON Toolbox
  Gain : Gain  Gain=cPhi1
  Gain1 : Gain  Gain=cPhi2
  Power : Math  Operator=pow
  Power1 : Math  Operator=pow
  Sign : Signum
  Sum1 : Sum  Inputs=+-
  Sum2 : Sum  Inputs=+++
  Sum3 : Sum  Inputs=+-
  S2 : Outport  VectorParamsAs1DForOutWhenUnconnected=off
  wires:
  xd2/1 -> Sum1/2
  Sum2/1 -> S2/1
  xd1/1 -> Sum3/2
  x1/1 -> Sum3/1
  x2/1 -> Sum1/1
  Sum3/1 -> Power1/1, Sign/1, Power/1
  Constant/1 -> Power/2
  Power/1 -> Gain/1
  Gain/1 -> Fractional integrator/1
  Constant1/1 -> Power1/2
  Sign/1 -> Divide/1
  Power1/1 -> Divide/2
  Divide/1 -> Gain1/1
  Gain1/1 -> Fractional integrator1/1
  Sum1/1 -> Sum2/1
  Fractional integrator/1 -> Sum2/2
  Fractional integrator1/1 -> Sum2/3

== system RobustFormationControl_FractionalModel_under_Dis/Fractional Leader with four followers/Follower 1 System/Follower 1 Quadrotor Model/Control Module1/Subsystem1/Subsystem1 ==
  x5 : Inport
  xd5 : Inport  Port=2
  x6 : Inport  Port=3
  xd6 : Inport  Port=4
  Constant : Constant  Value=p/q
  Constant1 : Constant  Value=gz
  Divide : Product  Inputs=**  RndMeth=Zero  SaturateOnIntegerOverflow=on
  Fractional integrator : fod/Fractional integrator  gam=alpha1(3)  ww=[0.001; 1000]  n=5  nFod=off
      settings: SourceProductName=FOMCON Toolbox
  Fractional integrator1 : fod/Fractional integrator  gam=alpha2(3)  ww=[0.001; 1000]  n=5  nFod=off
      settings: SourceProductName=FOMCON Toolbox
  Gain : Gain  Gain=cPsi1
  Gain1 : Gain  Gain=cPsi2
  Power : Math  Operator=pow
  Power1 : Math  Operator=pow
  Sign : Signum
  Sum1 : Sum  Inputs=+-
  Sum2 : Sum  Inputs=+++
  Sum3 : Sum  Inputs=+-
  S6 : Outport  VectorParamsAs1DForOutWhenUnconnected=off
  wires:
  xd6/1 -> Sum1/2
  Sum2/1 -> S6/1
  xd5/1 -> Sum3/2
  x5/1 -> Sum3/1
  x6/1 -> Sum1/1
  Sum3/1 -> Power1/1, Sign/1, Power/1
  Constant/1 -> Power/2
  Power/1 -> Gain/1
  Gain/1 -> Fractional integrator/1
  Constant1/1 -> Power1/2
  Sign/1 -> Divide/1
  Power1/1 -> Divide/2
  Divide/1 -> Gain1/1
  Gain1/1 -> Fractional integrator1/1
  Sum1/1 -> Sum2/1
  Fractional integrator/1 -> Sum2/2
  Fractional integrator1/1 -> Sum2/3

== system RobustFormationControl_FractionalModel_under_Dis/Fractional Leader with four followers/Follower 1 System/Follower 1 Quadrotor Model/Control Module1/Subsystem1/Subsystem2 ==
  yL : Inport
  x9 : Inport  Port=2
  x10 : Inport  Port=3
  dY : Inport  Port=4
  Constant : Constant  Value=p/q
  Constant1 : Constant  Value=gy
  Derivative : Derivative
  Derivative1 : Derivative
  Divide : Product  Inputs=**  RndMeth=Zero  SaturateOnIntegerOverflow=on
  Fractional integrator : fod/Fractional integrator  gam=alpha1(2)  ww=[0.001; 1000]  n=5  nFod=off
      settings: SourceProductName=FOMCON Toolbox
  Fractional integrator1 : fod/Fractional integrator  gam=alpha2(2)  ww=[0.001; 1000]  n=5  nFod=off
      settings: SourceProductName=FOMCON Toolbox
  Gain2 : Gain  Gain=cy1
  Gain3 : Gain  Gain=cy2
  Power : Math  Operator=pow
  Power1 : Math  Operator=pow
  Sign : Signum
  Sum1 : Sum  Inputs=+--
  Sum3 : Sum  Inputs=+--
  Sum5 : Sum  Inputs=+++
  S10 : Outport  VectorParamsAs1DForOutWhenUnconnected=off
  wires:
  x9/1 -> Sum3/2
  yL/1 -> Sum3/1, Derivative/1
  dY/1 -> Sum3/3, Derivative1/1
  x10/1 -> Sum1/3
  Derivative/1 -> Sum1/1
  Derivative1/1 -> Sum1/2
  Fractional integrator1/1 -> Sum5/3
  Fractional integrator/1 -> Sum5/2
  Gain3/1 -> Fractional integrator1/1
  Sum1/1 -> Sum5/1
  Sum5/1 -> S10/1
  Divide/1 -> Gain3/1
  Gain2/1 -> Fractional integrator/1
  Sign/1 -> Divide/1
  Power1/1 -> Divide/2
  Power/1 -> Gain2/1
  Constant1/1 -> Power1/2
  Sum3/1 -> Power1/1, Sign/1, Power/1
  Constant/1 -> Power/2

== system RobustFormationControl_FractionalModel_under_Dis/Fractional Leader with four followers/Follower 1 System/Follower 1 Quadrotor Model/Control Module1/Subsystem1/Subsystem3 ==
  xL : Inport
  x7 : Inport  Port=2
  x8 : Inport  Port=3
  dX : Inport  Port=4
  Constant : Constant  Value=p/q
  Constant1 : Constant  Value=gx
  Derivative : Derivative
  Derivative1 : Derivative
  Divide : Product  Inputs=**  RndMeth=Zero  SaturateOnIntegerOverflow=on
  Fractional integrator : fod/Fractional integrator  gam=alpha1(1)  ww=[0.001; 1000]  n=5  nFod=off
      settings: SourceProductName=FOMCON Toolbox
  Fractional integrator1 : fod/Fractional integrator  gam=alpha2(1)  ww=[0.001; 1000]  n=5  nFod=off
      settings: SourceProductName=FOMCON Toolbox
  Gain2 : Gain  Gain=cx1
  Gain3 : Gain  Gain=cx2
  Power : Math  Operator=pow
  Power1 : Math  Operator=pow
  Sign : Signum
  Sum1 : Sum  Inputs=+--
  Sum3 : Sum  Inputs=+--
  Sum5 : Sum  Inputs=+++
  S8 : Outport  VectorParamsAs1DForOutWhenUnconnected=off
  wires:
  x7/1 -> Sum3/2
  xL/1 -> Sum3/1, Derivative/1
  dX/1 -> Sum3/3, Derivative1/1
  x8/1 -> Sum1/3
  Derivative/1 -> Sum1/1
  Derivative1/1 -> Sum1/2
  Fractional integrator1/1 -> Sum5/3
  Fractional integrator/1 -> Sum5/2
  Gain3/1 -> Fractional integrator1/1
  Sum1/1 -> Sum5/1
  Sum5/1 -> S8/1
  Divide/1 -> Gain3/1
  Gain2/1 -> Fractional integrator/1
  Sign/1 -> Divide/1
  Power1/1 -> Divide/2
  Power/1 -> Gain2/1
  Constant1/1 -> Power1/2
  Sum3/1 -> Power1/1, Sign/1, Power/1
  Constant/1 -> Power/2
